simulink model "scheme"  (R2025a)
settings: Solver=ode45  StartTime=0.0  StopTime=10  MaxStep=0.005  RelTol=1e-3
settings Model: Creator=maksim  LastModifiedBy=maksim

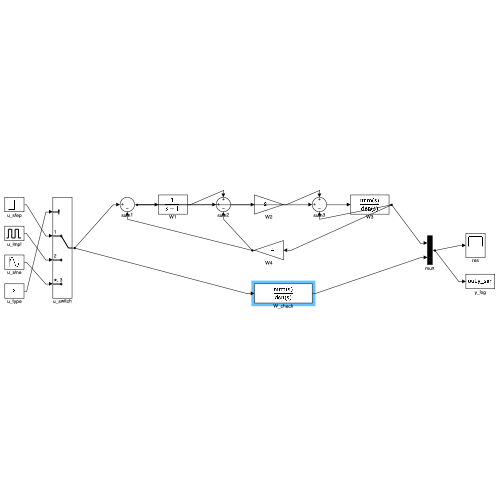
[thumbnail: Simulink's stored preview of the top-level diagram]
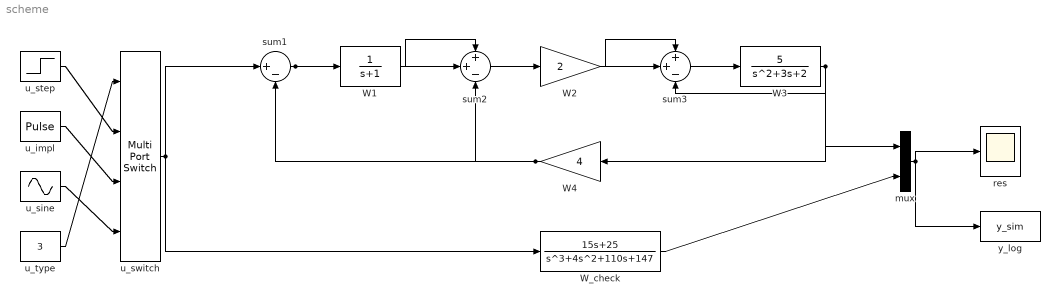
== system scheme ==
  W1 : TransferFcn  Denominator=[1 1]
  W2 : Gain  Gain=2
  W3 : TransferFcn  Numerator=[5]  Denominator=[1 3 2]
  W4 : Gain  Gain=4
  W_check : TransferFcn  Numerator=[15 25]  Denominator=[1 4 110 147]
  mux : Mux  Inputs=2
  res : Scope
      settings: ActiveDisplayYMinimum=-0.19602806634532624  ActiveDisplayYMaximum=0.19724147388468974
  sum1 : Sum  Inputs=|+-
  sum2 : Sum  Inputs=++-
  sum3 : Sum  Inputs=++-
  u_impl : DiscretePulseGenerator  PulseType=Time based  Amplitude=10  Period=10  PhaseDelay=1
  u_sine : Sin  Frequency=2  SampleTime=0
  u_step : Step  SampleTime=0
  u_switch : MultiPortSwitch  SaturateOnIntegerOverflow=off  InputSameDT=off
  u_type : Constant  Value=3
  y_log : ToWorkspace  VariableName=y_sim  SampleTime=-1
  wires:
  u_type/1 -> u_switch/1
  u_step/1 -> u_switch/2
  u_impl/1 -> u_switch/3
  u_sine/1 -> u_switch/4
  u_switch/1 -> sum1/1, W_check/1
  sum1/1 -> W1/1, sum2/2, sum3/2
  W1/1 -> sum2/1
  sum2/1 -> W2/1
  W2/1 -> sum3/1
  sum3/1 -> W3/1
  W3/1 -> sum3/3, W4/1, mux/1
  W4/1 -> sum1/2, sum2/3
  W_check/1 -> mux/2
  mux/1 -> res/1, y_log/1
